simulink model "simulationexo1"  (R2016a)
settings: Solver=VariableStepAuto  StartTime=0.0  StopTime=250  RelTol=1e-3
libraries: powerlib x1
settings Model: Creator=HP  LastModifiedBy=HP

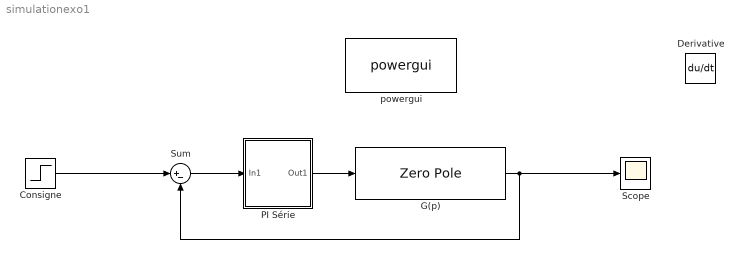
== system simulationexo1 ==
  "Consigne " : Step  Time=0  SampleTime=2e-6
  Derivative : Derivative
  "G(p) " : ZeroPole  Zeros=[]  Poles=[-1/5 -1/5 -1/5 -1/5]  Gain=[10/5^4]
  "PI Série " : Subsystem
  Scope : Scope
  Sum : Sum  Inputs=|+-
  powergui : powerlib/powergui  Priority=1  SimulationMode=Discrete  SolverType=Tustin/Backward Euler (TBE)  SampleTime=2e-6  frequency=60  SPID=off  DisableSnubberDevices=off  DisableRonSwitches=off  DisableVfSwitches=off  SwTol=0  DisplayEquations=off  Interpol=off  ExternalGateDelay=off  methode=off  Ts=10  FunctionMessages=off  echomessages=off  HookPort=off  EnableUseOfTLC=off  x0status=blocks  frequencyindice=60  Pbase=100e6  ErrMax=1e-4  Iterations=50  UnitsV=kV  UnitsW=MW  buscounter=0  RestoreLinks=warning  ResistiveCurrentMeasurement=off  Frange=[0:2:500]  Ylog=off  Xlog=on  ShowGrid=off  save=off  variable=ZData  structure=0  ZoomFFT=off  StartTime=0.0  cycles=1  DisplayStyle=1  fundamental=60  FreqAxis=off  MaxFrequency=1000  frequencyindicesteady=1  RmsSteady=1  display=off
  wires:
  "G(p) "/1 -> Scope/1, Sum/2
  "Consigne "/1 -> Sum/1
  Sum/1 -> "PI Série "/1(In1)
  "PI Série "/1(Out1) -> "G(p) "/1

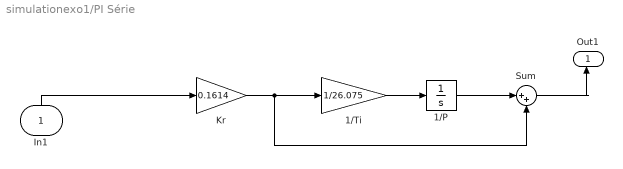
== system simulationexo1/PI Série  ==
  In1 : Inport
  "1/P " : Integrator
  "1/Ti " : Gain  Gain=1/26.075
  "Kr " : Gain  Gain=0.1614
  Sum : Sum  Inputs=|++
  Out1 : Outport
  wires:
  "1/Ti "/1 -> "1/P "/1
  "Kr "/1 -> "1/Ti "/1, Sum/2
  "1/P "/1 -> Sum/1
  Sum/1 -> Out1/1
  In1/1 -> "Kr "/1
